simulink model "third_order_MASH"  (R2022b)
settings: Solver=VariableStepAuto  StartTime=0.0  StopTime=0.32  RelTol=1e-3
libraries: dspsrcs4 x1
settings Model: Creator=khaled  LastModifiedBy=khaled
settings OptimizationCC: ReuseModelBlockBuffer=on
settings RTWCC: GPUComputeCapability=5.0

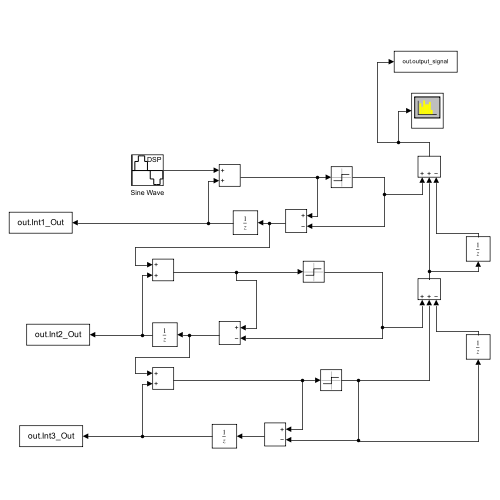
[thumbnail: Simulink's stored preview of the top-level diagram]
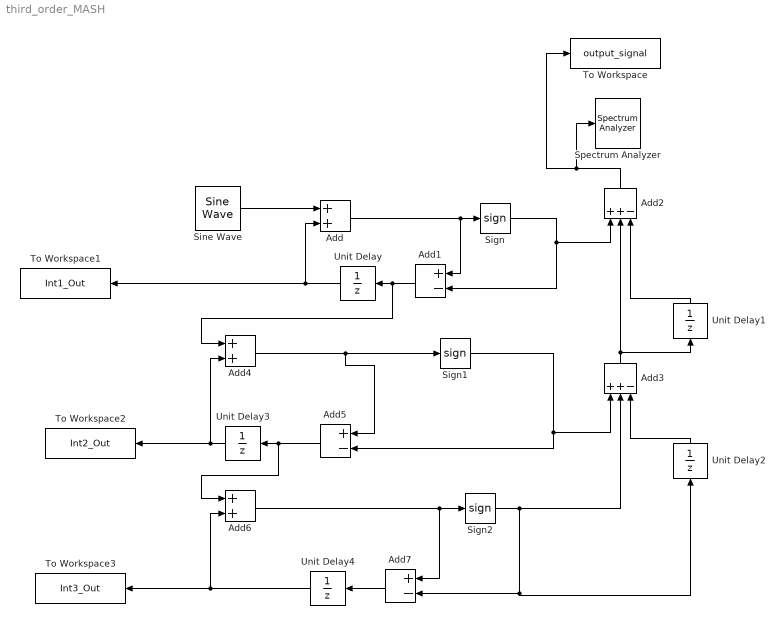
== system third_order_MASH ==
  Add : Sum
  Add1 : Sum  Inputs=+-
  Add2 : Sum  Inputs=++-
  Add3 : Sum  Inputs=++-
  Add4 : Sum
  Add5 : Sum  Inputs=+-
  Add6 : Sum
  Add7 : Sum  Inputs=+-
  Sign : Signum
  Sign1 : Signum
  Sign2 : Signum
  Sine Wave : dspsrcs4/Sine Wave  Amplitude=1  Frequency=100e3  Phase=0  SampleMode=Discrete  OutComplex=Real  CompMethod=Trigonometric fcn  TableSize=Speed  SampleTime=1e-8  SamplesPerFrame=1  ResetState=Restart at time zero  OutputFrames=off  dataType=double  wordLen=16  udDataType=sfix(16)  fracBitsMode=Best precision  numFracBits=15  OutDataTypeStr=double  LastOutDataTypeStr=double
  Spectrum Analyzer : SpectrumAnalyzer  DefaultConfigurationName=spbscopes.SpectrumAnalyzerBlockCfg
  To Workspace : ToWorkspace  VariableName=output_signal  SaveFormat=Timeseries  SampleTime=-1
  To Workspace1 : ToWorkspace  VariableName=Int1_Out  SaveFormat=Timeseries  SampleTime=-1
  To Workspace2 : ToWorkspace  VariableName=Int2_Out  SaveFormat=Timeseries  SampleTime=-1
  To Workspace3 : ToWorkspace  VariableName=Int3_Out  SaveFormat=Timeseries  SampleTime=-1
  Unit Delay{,1..4} (5 alike) : UnitDelay  SampleTime=-1  HasFrameUpgradeWarning=on
  wires:
  Sine Wave/1 -> Add/1
  Unit Delay/1 -> To Workspace1/1, Add/2
  Add/1 -> Add1/1, Sign/1
  Sign/1 -> Add1/2, Add2/1
  Add2/1 -> To Workspace/1, Spectrum Analyzer/1
  Unit Delay1/1 -> Add2/3
  Add3/1 -> Unit Delay1/1, Add2/2
  Unit Delay2/1 -> Add3/3
  Add5/1 -> Add6/1, Unit Delay3/1
  Sign1/1 -> Add3/1, Add5/2
  Add4/1 -> Add5/1, Sign1/1
  Add1/1 -> Add4/1, Unit Delay/1
  Unit Delay3/1 -> To Workspace2/1, Add4/2
  Add7/1 -> Unit Delay4/1
  Sign2/1 -> Add3/2, Unit Delay2/1, Add7/2
  Add6/1 -> Add7/1, Sign2/1
  Unit Delay4/1 -> To Workspace3/1, Add6/2
